simulink model "dc_fed_grid_connected_vsi_open_loop"  (R2025a)
settings: Solver=FixedStepAuto  StartTime=0.0  StopTime=0.1  FixedStep=1e-5  RelTol=1e-3
libraries: spsDCVoltageSourceLib x1, eePwmGeneratorTwoLevel x1, spsThreePhaseSeriesRLCBranchLib x1, spsThreePhaseVIMeasurementLib x1, spsThreePhaseSourceLib x1, spsUniversalBridgeLib x1, spsVoltageMeasurementLib x1, sps_lib x1
settings Model: Creator=HAKAN SARI  LastModifiedBy=HAKAN SARI

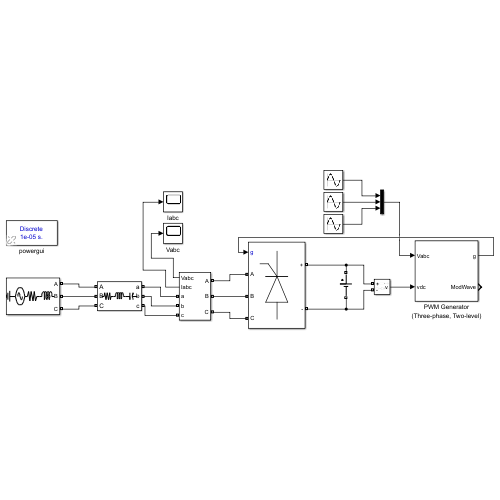
[thumbnail: Simulink's stored preview of the top-level diagram]
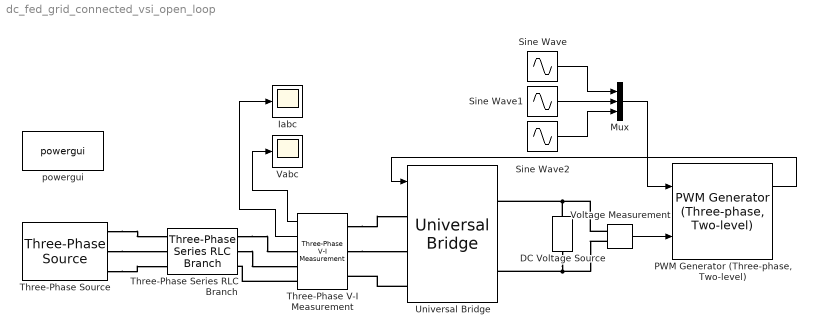
== system dc_fed_grid_connected_vsi_open_loop ==
  DC Voltage Source : spsDCVoltageSourceLib/DC Voltage Source  Amplitude=700  Measurements=None
  Iabc : Scope
      settings: ActiveDisplayYMinimum=-0.0081648678196405387  ActiveDisplayYMaximum=0.0081648678196408683
  Mux : Mux  Inputs=3
  "PWM Generator (Three-phase, Two-level)" : eePwmGeneratorTwoLevel/PWM Generator (Three-phase, Two-level)  PWMMode=Continuous PWM (CPWM)  CPWMMode=SPWM: sinusoidal PWM  DPWMMode=60 DPWM: 60 degree discontinuous PWM  fsw=5e3  Ts=1e-5
      settings: LibrarySourceBlock=|
      | ee_sl_lib/Pulse Width
      | Modulation/PWM Generator
      | (Three-phase, Two-level)
  Sine Wave : Sin  Amplitude=0.5  Frequency=314.159  SampleTime=0
  Sine Wave1 : Sin  Amplitude=0.5  Frequency=314.159  Phase=-2*pi/3  SampleTime=0
  Sine Wave2 : Sin  Amplitude=0.5  Frequency=314.159  Phase=2*pi/3  SampleTime=0
  Three-Phase Series RLC Branch : spsThreePhaseSeriesRLCBranchLib/Three-Phase Series RLC Branch  LConnTagsString=A|B|C  RConnTagsString=A|B|C  BranchType=RLC  Resistance=0.5  Inductance=5e-3  Capacitance=0  Measurements=None
  Three-Phase V-I Measurement : spsThreePhaseVIMeasurementLib/Three-Phase V-I Measurement  VoltageMeasurement=phase-to-ground  SetLabelV=off  LabelV=Vabc  Vpu=off  VpuLL=off  CurrentMeasurement=yes  SetLabelI=off  LabelI=Iabc  Ipu=off  Pbase=100e6  Vbase=500e3  OutputType=Complex  PhasorSimulation=off  PSBequivalent=0
  Three-Phase Source : spsThreePhaseSourceLib/Three-Phase Source  InternalConnection=Yg  VoltagePhases=off  Voltage=400  PhaseAngle=0  Voltage_phases=[25e3 25e3 25e3]/sqrt(3)  PhaseAngles_phases=[0 -120 +120]  Frequency=50  NonIdealSource=on  SpecifyImpedance=off  Resistance=0.1  Inductance=1e-3  ShortCircuitLevel=100e6  BaseVoltage=400  XRratio=7  BusType=swing  Pref=10e3  Qref=0  Prefabc=[10e3, 10e3, 10e3]  Qrefabc=[0, 0, 0]  Qmin=-inf  Qmax=inf
  Universal Bridge : spsUniversalBridgeLib/Universal Bridge  Arms=3  SnubberResistance=1e5  SnubberCapacitance=inf  Device=Thyristors  Ron=1e-3  Lon=0  ForwardVoltages="[  0  0  ]"  ForwardVoltage=0  GTOparameters=[ 10e-6 , 20e-6 ]  IGBTparameters=[ 1e-6 , 2e-6 ]  Measurements=None  Measurements_2=None  converterType=Rectifier
  Vabc : Scope
      settings: ActiveDisplayYMinimum=-408.24339098200716  ActiveDisplayYMaximum=408.24339098202279
  Voltage Measurement : spsVoltageMeasurementLib/Voltage Measurement  PhasorSimulation=off  OutputType=Complex  PSBequivalent=0
  powergui : sps_lib/powergui  Priority=1  SimulationMode=Discrete  SampleTime=1e-5  frequency=60  Iterations=50  frequencyindice=50  Pbase=100e6  ErrMax=1e-4  UnitsV=kV  UnitsW=MW  buscounter=0  FunctionMessages=off  echomessages=off  EnableUseOfTLC=off  CurrentSourceSwitches=off  DisableSnubberDevices=off  DisableRonSwitches=off  DisableVfSwitches=off  DisplayEquations=off  AutomaticDiscreteSolvers=off  SolverType=Tustin/Backward Euler (TBE)  Interpol=off  ExternalGateDelay=off  methode=off  Ts=100  x0status=blocks  SPID=on  SwTol=0  HookPort=off  NonlinearTolerance=1e-4  nMaxIteration=100  ContinueOnMaxIteration=off  RestoreLinks=warning  ResistiveCurrentMeasurement=off  Frange=[0:2:500]  Ylog=off  Xlog=on  ShowGrid=off  save=off  variable=ZData  structure=0  ZoomFFT=off  StartTime=0.0  cycles=1  DisplayStyle=1  fundamental=60  FreqAxis=off  MaxFrequency=1000  frequencyindicesteady=1  RmsSteady=1  display=off
  wires:
  Voltage Measurement/1 -> "PWM Generator (Three-phase, Two-level)"/2
  Sine Wave/1 -> Mux/1
  Sine Wave1/1 -> Mux/2
  Sine Wave2/1 -> Mux/3
  Mux/1 -> "PWM Generator (Three-phase, Two-level)"/1
  "PWM Generator (Three-phase, Two-level)"/1 -> Universal Bridge/1
  Three-Phase V-I Measurement/1 -> Vabc/1
  Three-Phase V-I Measurement/2 -> Iabc/1
  connections:
  DC Voltage Source/RConn1 -- Voltage Measurement/LConn1 -- Universal Bridge/RConn1
  DC Voltage Source/LConn1 -- Voltage Measurement/LConn2 -- Universal Bridge/RConn2
  Three-Phase Source/RConn1 -- Three-Phase Series RLC Branch/LConn1
  Three-Phase Source/RConn2 -- Three-Phase Series RLC Branch/LConn2
  Three-Phase Source/RConn3 -- Three-Phase Series RLC Branch/LConn3
  Three-Phase Series RLC Branch/RConn1 -- Three-Phase V-I Measurement/RConn1
  Three-Phase Series RLC Branch/RConn2 -- Three-Phase V-I Measurement/RConn2
  Three-Phase V-I Measurement/RConn3 -- Three-Phase Series RLC Branch/RConn3
  Three-Phase V-I Measurement/LConn1 -- Universal Bridge/LConn1
  Three-Phase V-I Measurement/LConn2 -- Universal Bridge/LConn2
  Universal Bridge/LConn3 -- Three-Phase V-I Measurement/LConn3
